simulink model "microgrid_pv_batterie"  (R2024a)
settings: Solver=VariableStepAuto  StartTime=0.0  StopTime=10.0  RelTol=1e-3
undefined symbols (not defined in the file): Ion, Lithium
libraries: spsSeriesRLCBranchLib x5, spsMosfetLib x3, spsPWMGeneratorDCDCLib x2, spsBatteryLib x1, spsCurrentMeasurementLib x1, spsDiodeLib x1, slpidlib x1, spsPVArrayLib x1, simulink x1, spsVoltageMeasurementLib x1, sps_lib x1
settings Model: Creator=Najoua  LastModifiedBy=hp

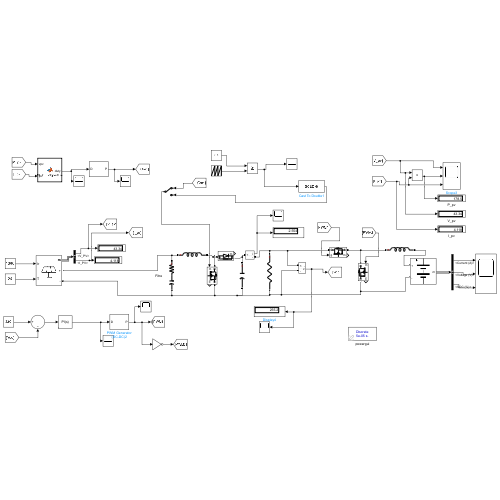
[thumbnail: Simulink's stored preview of the top-level diagram]
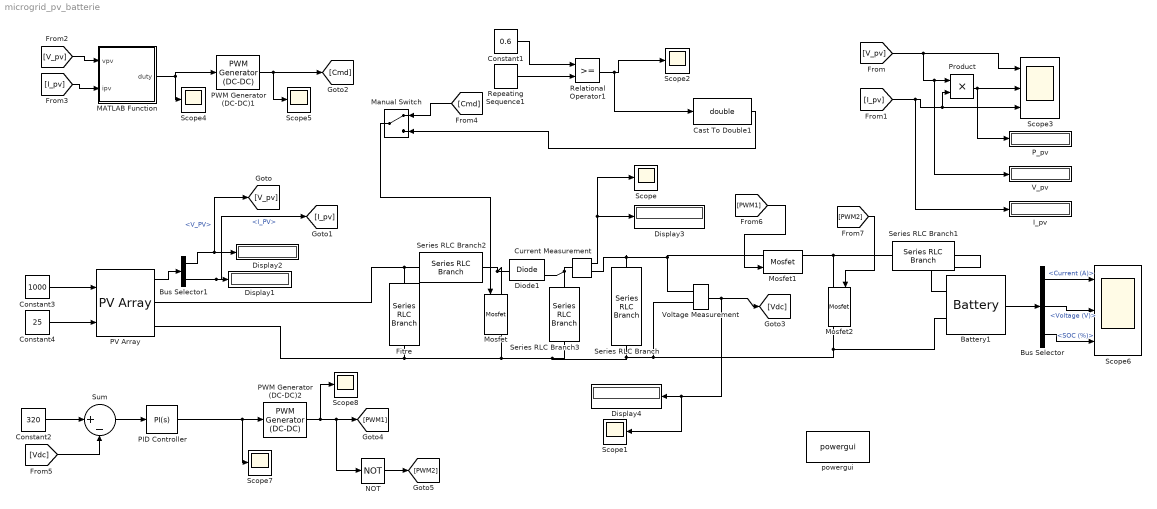
== system microgrid_pv_batterie ==
  Battery1 : spsBatteryLib/Battery  BatType=Lithium-Ion  ShowTempParam=off  ThermalPreset=no  ShowAgeParam=off  NomV=320  NomQ=5.4  SOC=100  Batt_Tr=30  PresetModel=on  MaxQ=5.4  MinV=240  FullV=372.4759  Dis_rate=2.3478  R=0.59259  Normal_OP=4.8835  expZone="[345.7235     0.2653043]"  current=[6.5 13 32.5]  Units=Time  Tci=20  NomT=20  T2=-30  MaxQ2=4.8  FullV2=7.1  Normal_OP2=5.655  expZone2="[6.58           1]"  Rca=0.6  ti=2000  Dp=0  Neq0=0  Tsim=1e6  Ta1=25  Qeol=5.4*0.9  Reol=0.013333*1.2  Char_age=[2.3478, 3]  Dis_age=[2.3478, 10]  N1=1500  N2=10500  N3=1000  N4=1400  Ta2=45  N5=950
  Bus Selector : BusSelector  OutputSignals=Current (A),Voltage (V),SOC (%)
  Bus Selector1 : BusSelector  OutputSignals=V_PV,I_PV
  Cast To Double1 : DataTypeConversion  OutMax=[12]  OutDataTypeStr=double  SaturateOnIntegerOverflow=off  RndMeth=Floor
  Constant1 : Constant  Value=0.6
  Constant2 : Constant  Value=320
  Constant3 : Constant  Value=1000
  Constant4 : Constant  Value=25
  Current Measurement : spsCurrentMeasurementLib/Current Measurement  PhasorSimulation=off  OutputType=Complex  PSBequivalent=0
  Diode1 : spsDiodeLib/Diode  Ron=0.001  Lon=0  Vf=0.8  IC=0  UseSnubber=0  Rs=500  Cs=250e-9  Measurements=on
  Display{1..4} (4 alike) : Display
  "Fitre " : spsSeriesRLCBranchLib/Series RLC Branch  LConnTagsString=__new0  RConnTagsString=__new0  BranchType=RC  Resistance=0.0001  Inductance=1e-3  SetiL0=off  InitialCurrent=0  Capacitance=1.66e-4  Setx0=off  InitialVoltage=0  Measurements=None
  I_pv : Display
  MATLAB Function : MATLAB Function  TreatAsAtomicUnit=on
  Manual Switch : ManualSwitch
  Mosfet : spsMosfetLib/Mosfet  Ron=0.1  Lon=0  Rd=0.01  Vfd=0  IC=0  Rs=1e5  Cs=inf  Measurements=on
  Mosfet1 : spsMosfetLib/Mosfet  Ron=0.1  Lon=0  Rd=0.01  Vfd=0  IC=0  Rs=1e5  Cs=inf  Measurements=on
  Mosfet2 : spsMosfetLib/Mosfet  Ron=0.1  Lon=0  Rd=0.01  Vfd=0  IC=0  Rs=1e5  Cs=inf  Measurements=on
  NOT : Logic  Operator=NOT  IconShape=distinctive  AllPortsSameDT=off  OutDataTypeStr=boolean
  PID Controller : slpidlib/PID Controller  Controller=PI  Form=Parallel  TimeDomain=Continuous-time  UseExternalTs=off  SampleTime=-1  IntegratorMethod=Forward Euler  FilterMethod=Forward Euler  ControllerParametersSource=internal  P=1  I=10  UseKiTs=off  D=0  UseExternalDerivativeSource=off  N=100  UseFilter=on  TunerSelectOption=Transfer Function Based (PID Tuner App)  InitialConditionSource=internal  InitialConditionForIntegrator=0  InitialConditionForFilter=0  DifferentiatorICPrevScaledInput=0  ExternalReset=none  TrackingMode=off  Kt=1  LimitOutput=off  SatLimitsSource=internal  UpperSaturationLimit=inf  LowerSaturationLimit=-inf  LinearizeAsGain=on  AntiWindupMode=none  Kb=1  LimitIntegrator=off  UpperIntegratorSaturationLimit=inf  LowerIntegratorSaturationLimit=-inf  POutMin=[]  POutMax=[]  IOutMin=[]  IOutMax=[]  DOutMin=[]  DOutMax=[]  NOutMin=[]  NOutMax=[]  SumOutMin=[]  SumOutMax=[]  SaturationOutMin=[]  SaturationOutMax=[]  PParamMin=[]  PParamMax=[]  IParamMin=[]  IParamMax=[]  DParamMin=[]  DParamMax=[]  NParamMin=[]  NParamMax=[]  KbParamMin=[]  KbParamMax=[]  KtParamMin=[]  KtParamMax=[]  KbOutMin=[]  KbOutMax=[]  KtOutMin=[]  KtOutMax=[]  IntegratorOutMin=[]  IntegratorOutMax=[]  FilterOutMin=[]  FilterOutMax=[]  SumI1OutMin=[]  SumI1OutMax=[]  SumI2OutMin=[]  SumI2OutMax=[]  SumI3OutMin=[]  SumI3OutMax=[]  SumI4OutMin=[]  SumI4OutMax=[]  SumDOutMin=[]  SumDOutMax=[]  DifferentiatorOutMin=[]  DifferentiatorOutMax=[]  FilterDiffOutCoefMin=[]  FilterDiffOutCoefMax=[]  ReciprocalOutMin=[]  ReciprocalOutMax=[]  SumDenOutMin=[]  SumDenOutMax=[]  SumNumOutMin=[]  SumNumOutMax=[]  DivideOutMin=[]  DivideOutMax=[]  UdiffTsProdOutMin=[]  UdiffTsProdOutMax=[]  NTsProdOutMin=[]  NTsProdOutMax=[]  UintegralTsProdOutMin=[]  UintegralTsProdOutMax=[]  UngainTsProdOutMin=[]  UngainTsProdOutMax=[]  ClampingZeroOutDataTypeStr=Inherit: Inherit via back propagation  ClampingZeroOutMin=[]  ClampingZeroOutMax=[]  FilterDenConstantOutDataTypeStr=Inherit: Inherit via back propagation  FilterDenConstantOutMin=[]  FilterDenConstantOutMax=[]  PCopyOutDataTypeStr=Inherit: Inherit via back propagation  PCopyOutMin=[]  PCopyOutMax=[]  NCopyOutDataTypeStr=Inherit: Inherit via back propagation  NCopyOutMin=[]  NCopyOutMax=[]  IntegratorContinuousStateAttributes=''  IntegratorStateMustResolveToSignalObject=off  IntegratorRTWStateStorageClass=Auto  FilterContinuousStateAttributes=''  FilterStateMustResolveToSignalObject=off  FilterRTWStateStorageClass=Auto  ParallelPVariant=InternalParameters  IdealPVariant=Disabled  IVariant=InternalParameters  DVariant=Disabled  IntegratorVariant=Continuous  SatVariant=Disabled  AWVariant=Passthrough  PCopyVariant=Disabled  TRVariant=Disabled  FdbkBlocksVariant=Forward  IdealPFdbkVariant=Disabled  SatFdbkVariant=Disabled  DerivativeFilterVariant=Disabled  NVariant=Disabled  NCopyVariant=Disabled_SignalSpec  FilterICVariant=Disabled  IntegratorICVariant=InternalICs  ExternalResetVariant=Disabled  TRSumVariant=Passthrough  SumFdbkVariant=Disabled  SumVariant=Sum_PI  TsampFilterVariant=InternalTs  TsampNgainVariant=Passthrough  TsampIntegralVariant=Disabled_SignalSpec  ExternalSaturationOutDataTypeStr=Inherit: Same as second input  DerivativeSourceVariant=Disabled
  PV Array : spsPVArrayLib/PV Array  Npar=1  Nser=1  PlotType=array @ 25 deg.C & specified irradiances  S_vec="[ 1000  500  100 ]"  Temp_C_vec="[ 45 25  ]"  ModuleName=A10Green Technology A10J-S72-175  PlotWhenSelected=off  Pm=175.0914  Ncell=72  Voc=43.99  Isc=5.17  Vm=36.63  Im=4.78  beta_Voc_pc=-0.3616  alpha_Isc_pc=0.041509  beta_Voc=-0.15907  alpha_Isc=0.002146  IL=5.178  I0=1.7842e-10  nI=0.98852  Rsh=249.6758  Rs=0.38412  RobustModel=off  RobustCellTemperature=313.3991  BAL=on  Tc=1e-6  Tfilter=5e-5
  PWM Generator (DC-DC)1 : spsPWMGeneratorDCDCLib/PWM Generator (DC-DC)  Fsw=10000  Ts=0
  PWM Generator (DC-DC)2 : spsPWMGeneratorDCDCLib/PWM Generator (DC-DC)  Fsw=5000  Ts=0
  P_pv : Display
  Product : Product
  Relational Operator1 : RelationalOperator  OutDataTypeStr=boolean  RndMeth=Simplest  InputSameDT=off
  Repeating Sequence1 : simulink/Sources/Repeating Sequence  rep_seq_t=[0 0.001]  rep_seq_y=[0 1 ]
  Scope{,1..2,4..5,7..8} (7 alike) : Scope
  Scope3 : Scope  NumInputPorts=3
  Scope6 : Scope  NumInputPorts=3
  Series RLC Branch : spsSeriesRLCBranchLib/Series RLC Branch  LConnTagsString=__new0  RConnTagsString=__new0  BranchType=R  Resistance=100  Inductance=1e-3  SetiL0=off  InitialCurrent=0  Capacitance=1e-6  Setx0=off  InitialVoltage=0  Measurements=None
  Series RLC Branch1 : spsSeriesRLCBranchLib/Series RLC Branch  LConnTagsString=__new0  RConnTagsString=__new0  BranchType=L  Resistance=1  Inductance=0.0025  SetiL0=off  InitialCurrent=0  Capacitance=1e-6  Setx0=off  InitialVoltage=0  Measurements=None
  Series RLC Branch2 : spsSeriesRLCBranchLib/Series RLC Branch  LConnTagsString=__new0  RConnTagsString=__new0  BranchType=L  Resistance=1  Inductance=0.0025  SetiL0=off  InitialCurrent=0  Capacitance=1e-6  Setx0=off  InitialVoltage=0  Measurements=None
  Series RLC Branch3 : spsSeriesRLCBranchLib/Series RLC Branch  LConnTagsString=__new0  RConnTagsString=__new0  BranchType=C  Resistance=1  Inductance=1e-3  SetiL0=off  InitialCurrent=0  Capacitance=18e-6  Setx0=off  InitialVoltage=0  Measurements=None
  Sum : Sum  Inputs=|+-
  V_pv : Display
  Voltage Measurement : spsVoltageMeasurementLib/Voltage Measurement  PhasorSimulation=off  OutputType=Complex  PSBequivalent=0
  powergui : sps_lib/powergui  Priority=1  SimulationMode=Discrete  SampleTime=50e-6  frequency=60  Iterations=50  frequencyindice=0  Pbase=100e6  ErrMax=1e-4  UnitsV=kV  UnitsW=MW  buscounter=0  FunctionMessages=off  echomessages=off  EnableUseOfTLC=off  CurrentSourceSwitches=off  DisableSnubberDevices=off  DisableRonSwitches=off  DisableVfSwitches=off  DisplayEquations=off  AutomaticDiscreteSolvers=off  SolverType=Tustin/Backward Euler (TBE)  Interpol=off  ExternalGateDelay=off  methode=off  Ts=100  x0status=blocks  SPID=on  SwTol=0  HookPort=off  NonlinearTolerance=1e-4  nMaxIteration=100  ContinueOnMaxIteration=off  RestoreLinks=warning  ResistiveCurrentMeasurement=off  Frange=[0:2:500]  Ylog=off  Xlog=on  ShowGrid=off  save=off  variable=ZData  structure=0  ZoomFFT=off  StartTime=0.0  cycles=1  DisplayStyle=1  fundamental=60  FreqAxis=off  MaxFrequency=1000  frequencyindicesteady=1  RmsSteady=1  display=off
  wires:
  Bus Selector1/2 -> [I_pv], Display1/1  "<I_PV>"
  PWM Generator (DC-DC)2/1 -> Scope8/1, NOT/1, [PWM1]
  [PWM1] -> Mosfet1/1
  [PWM2] -> Mosfet2/1
  PWM Generator (DC-DC)1/1 -> [Cmd], Scope5/1
  [I_pv] -> MATLAB Function/2(ipv)
  Repeating Sequence1/1 -> Relational Operator1/2
  Sum/1 -> PID Controller/1
  NOT/1 -> [PWM2]
  Current Measurement/1 -> Scope/1, Display3/1
  Bus Selector/3 -> Scope6/3  "<SOC (%)>"
  Relational Operator1/1 -> Scope2/1, Cast To Double1/1
  PID Controller/1 -> Scope7/1, PWM Generator (DC-DC)2/1
  [Cmd] -> Manual Switch/1
  Constant4/1 -> PV Array/2
  MATLAB Function/1(duty) -> PWM Generator (DC-DC)1/1, Scope4/1
  Bus Selector/1 -> Scope6/1  "<Current (A)>"
  [V_pv] -> V_pv/1, Product/1, Scope3/1
  Voltage Measurement/1 -> [Vdc], Scope1/1, Display4/1
  Cast To Double1/1 -> Manual Switch/2
  Constant2/1 -> Sum/1
  Battery1/1 -> Bus Selector/1
  [Vdc] -> Sum/2
  Constant3/1 -> PV Array/1
  [I_pv] -> I_pv/1, Product/2, Scope3/3
  Bus Selector/2 -> Scope6/2  "<Voltage (V)>"
  Bus Selector1/1 -> [V_pv], Display2/1  "<V_PV>"
  PV Array/1 -> Bus Selector1/1
  [V_pv] -> MATLAB Function/1(vpv)
  Constant1/1 -> Relational Operator1/1
  Product/1 -> P_pv/1, Scope3/2
  Manual Switch/1 -> Mosfet/1
  connections:
  Current Measurement/RConn1 -- Series RLC Branch/LConn1 -- Mosfet1/LConn1 -- Voltage Measurement/LConn1
  Voltage Measurement/LConn2 -- Mosfet2/RConn1 -- Battery1/LConn2 -- Mosfet/RConn1 -- "Fitre "/RConn1 -- PV Array/RConn2 -- Series RLC Branch3/RConn1 -- Series RLC Branch/RConn1
  PV Array/RConn1 -- "Fitre "/LConn1 -- Series RLC Branch2/LConn1
  Diode1/LConn1 -- Series RLC Branch2/RConn1 -- Mosfet/LConn1
  Mosfet2/LConn1 -- Mosfet1/RConn1 -- Series RLC Branch1/LConn1
  Series RLC Branch3/LConn1 -- Current Measurement/LConn1 -- Diode1/RConn1
  Battery1/LConn1 -- Series RLC Branch1/RConn1

== matlab function microgrid_pv_batterie/MATLAB Function ==
  settings: updateMethod=DISCRETE
  data: vpv input; duty output; ipv input
function duty =MPPT_algorithm(vpv,ipv) 
delta=0.1;
duty_min=0.1;
duty_max=0.9;

persistent Vold Pold duty_old;

if isempty(Vold)
    Vold=0;
    Pold=0; 
    duty_old=0;
end


P=vpv*ipv;

if P~= Pold
if (P-Pold)>0
if (vpv-Vold)>0 duty=duty_old -delta;
else
duty=duty_old +delta;
end 
else
if (vpv-Vold)>0 duty=duty_old +delta;
else
duty=duty_old -delta;
end
end
else
duty=duty_old ;
end

if duty>=duty_max
    duty=duty_max;

elseif duty<=duty_min
    duty=duty_min;
end

duty_old=duty;
Vold=vpv;
Pold=P;
